simulink model "sf_bus_operations"  (R2025b)
settings: Solver=FixedStepDiscrete  StartTime=0.0  StopTime=10.0  FixedStep=1  RelTol=1e-3  EnableMultiTasking=on
PostLoadFcn:
  | load myBuses
  | idx = 2;
settings Model: Creator=The MathWorks, Inc.  LastModifiedBy=The MathWorks, Inc.
settings SolverCC: AlgebraicLoopSolver=TrustRegion  MaxZcPerStep=1.0
settings DataIOCC: LimitDataPoints=on  SaveFormat=StructureWithTime  ReturnWorkspaceOutputs=off
settings OptimizationCC: ReuseModelBlockBuffer=off  ExpressionDepthLimit=2147483647.0  InitFltsAndDblsToZero=on  LifeSpan=inf
settings DebuggingCC: SaveWithParameterizedLinksMsg=none  UnderspecifiedInitializationDetection=Classic  MergeDetectMultiDrivingBlocksExec=none  SignalResolutionControl=TryResolveAllWithWarning  SolverPrmCheckMsg=warning  MultiTaskDSMMsg=warning  MultiTaskCondExecSysMsg=none  FcnCallInpInsideContextMsg=warning  UnconnectedInputMsg=warning  UnconnectedOutputMsg=warning  UnconnectedLineMsg=warning  StateNameClashWarn=warning  SFUnexpectedBacktrackingDiag=warning  SFNoUnconditionalDefaultTransitionDiag=warning  SFExecutionAtInitializationDiag=none  ArithmeticOperatorsInVariantConditions=warning
settings HardwareCC: ProdBitPerPointer=32.0  ProdBitPerSizeT=32.0  ProdBitPerPtrDiffT=32.0  ProdLargestAtomicFloat=None  ProdIntDivRoundTo=Undefined  ProdEndianess=Unspecified  ProdWordSize=32.0  ProdHWDeviceType=32-bit Generic
settings ModelReferenceCC: EnableRefExpFcnMdlSchedulingChecks=on  PropagateSignalLabelsOutOfModel=off
settings SFSimCC: SimUseLocalCustomCode=off  SimParseCustomCode=off  CustomCodeUndefinedFunction=UseInterfaceOnly
settings RTWCC: GenerateReport=on  RTWUseLocalCustomCode=off  LaunchReport=on  GPUComputeCapability=3.5  DLArmComputeVersion=19.05
settings CodeAppCC: StateflowObjectComments=on
settings GRTTargetCC: TargetFcnLib=ansi_tfl_tmw.mat  TargetLangStandard=C89/C90 (ANSI)  CombineOutputUpdateFcns=off  GRTInterface=on
settings ConfigComp: CovMetricSettings=dw  CovSaveCumulativeToWorkspaceVar=on  CovSaveSingleToWorkspaceVar=on  CovExternalEMLEnable=off

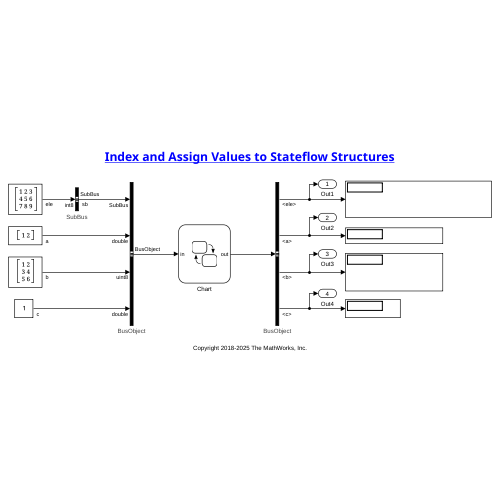
[thumbnail: Simulink's stored preview of the top-level diagram]
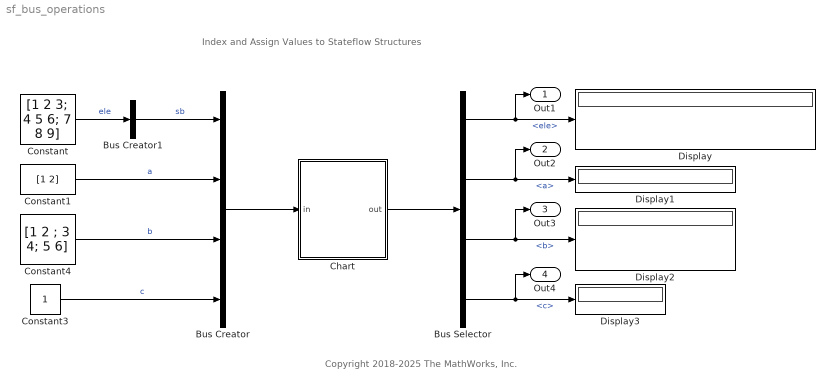
== system sf_bus_operations ==
  note: Copyright 2018-2025 The MathWorks, Inc.
  note: Index and Assign Values to Stateflow Structures
  Bus Creator : BusCreator  Inputs=4  OutDataTypeStr=Bus: BusObject  NonVirtualBus=on
      settings: AttributesFormatString=BusObject
  Bus Creator1 : BusCreator  Inputs=1  OutDataTypeStr=Bus: SubBus  NonVirtualBus=on
      settings: AttributesFormatString=SubBus
  Bus Selector : BusSelector  OutputSignals=sb.ele,a,b,c
      settings: AttributesFormatString=BusObject
  Chart : Stateflow chart  TreatAsAtomicUnit=on
  Constant : Constant  Value=[1 2 3; 4 5 6; 7 8 9]  OutDataTypeStr=int8
  Constant1 : Constant  Value=[1 2]  OutDataTypeStr=double
  Constant3 : Constant  OutDataTypeStr=double
  Constant4 : Constant  Value=[1 2 ; 3 4; 5 6]  OutDataTypeStr=uint8
  Display{,1..3} (4 alike) : Display
  Out1 : Outport  VectorParamsAs1DForOutWhenUnconnected=off
  Out2 : Outport  Port=2  VectorParamsAs1DForOutWhenUnconnected=off
  Out3 : Outport  Port=3  VectorParamsAs1DForOutWhenUnconnected=off
  Out4 : Outport  Port=4  VectorParamsAs1DForOutWhenUnconnected=off
  wires:
  Bus Creator/1 -> Chart/1(in)
  Bus Creator1/1 -> Bus Creator/1  "sb"
  Constant1/1 -> Bus Creator/2  "a"
  Constant3/1 -> Bus Creator/4  "c"
  Chart/1(out) -> Bus Selector/1
  Bus Selector/1 -> Display/1, Out1/1  "<ele>"
  Bus Selector/2 -> Display1/1, Out2/1  "<a>"
  Bus Selector/3 -> Out3/1, Display2/1  "<b>"
  Bus Selector/4 -> Display3/1, Out4/1  "<c>"
  Constant/1 -> Bus Creator1/1  "ele"
  Constant4/1 -> Bus Creator/3  "b"

== stateflow chart sf_bus_operations/Chart ==
  state A
    en:
    localbus = sb2abc(in.sb);
    subBusArray(1) = in.sb;
    subBusArray(2) = abc2sb(in);
    subBusArray(3).ele = transpose(in.sb.ele);
    subBusArray(4).ele = int8(magic(3));
    out = localbus;
    out.sb = subBusArray(idx);
  state y = abc2sb(u) [function]
    (default) -> (junction 6) : {
        | y.ele = int8([u.a(1) u.a(2) u.c; transpose(u.b)]);
        | }
  (default) -> A
  data: y function_output Bus: BusObject size=1; u function_input Bus: SubBus size=1; u function_input Bus: BusObject size=1; y function_output Bus: SubBus size=1; in input; out output Bus: BusObject size=1; subBusArray local Bus: SubBus size=4; localbus local Bus: BusObject size=1; idx parameter
  function y = sb2abc(u):
    | function y = sb2abc(u)
    | 
    | % extract data from input structure
    | 
    | A = double(u.ele(1:2,1));
    | B = uint8(u.ele(:,2:3));
    | C = double(u.ele(3,1));
    | 
    | % create local structure
    | 
    | X = struct(ele=int8(zeros(3)));
    | Y = struct(sb=X,a=A,b=B,c=C);
    | 
    | % assign value to output structure
    | 
    | y = Y;
    | 
    | end
